simulink model "WiperSystem"  (R2023b)
settings: Solver=VariableStepAuto  StartTime=0.0  StopTime=20  RelTol=1e-3
libraries: simulink x6
settings Model: Creator=SEIF  LastModifiedBy=SEIF

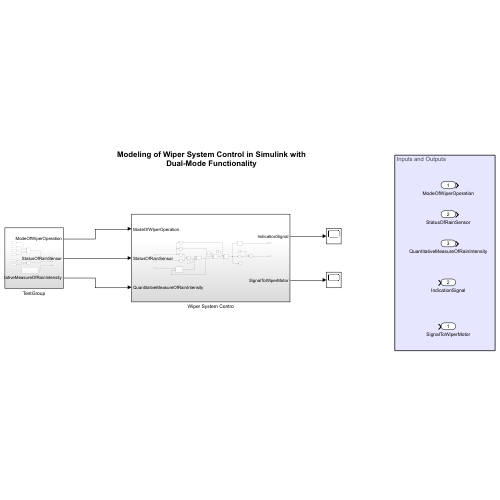
[thumbnail: Simulink's stored preview of the top-level diagram]
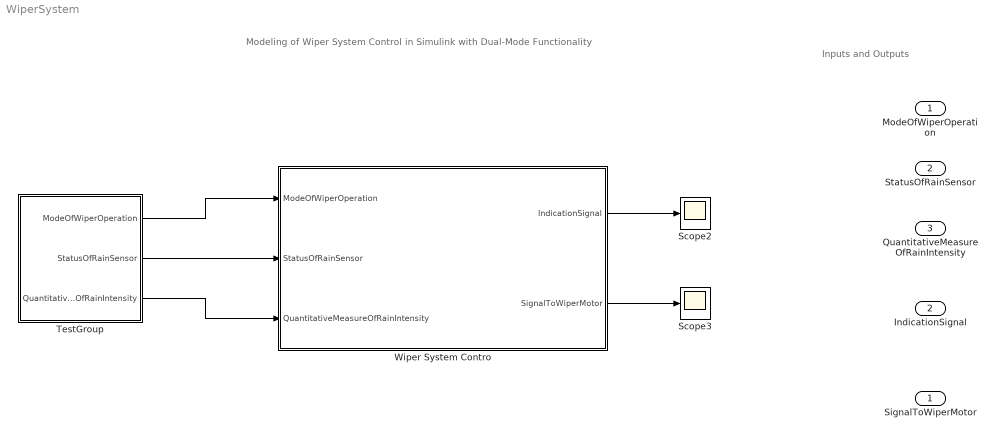
== system WiperSystem ==
  note: Inputs and Outputs
  note: Modeling of Wiper System Control in Simulink with Dual-Mode Functionality
  ModeOfWiperOperation : Inport
  StatusOfRainSensor : Inport  Port=2
  "QuantitativeMeasureOfRainIntensity " : Inport  Port=3
  Scope2 : Scope
  Scope3 : Scope
  TestGroup : Subsystem
  Wiper System Contro : Subsystem
  SignalToWiperMotor : Outport
  IndicationSignal : Outport  Port=2
  wires:
  TestGroup/3(QuantitativeMeasureOfRainIntensity) -> Wiper System Contro/3("QuantitativeMeasureOfRainIntensity ")
  TestGroup/2(StatusOfRainSensor) -> Wiper System Contro/2(StatusOfRainSensor)
  TestGroup/1(ModeOfWiperOperation) -> Wiper System Contro/1(ModeOfWiperOperation)
  Wiper System Contro/1(IndicationSignal) -> Scope2/1
  Wiper System Contro/2(SignalToWiperMotor) -> Scope3/1

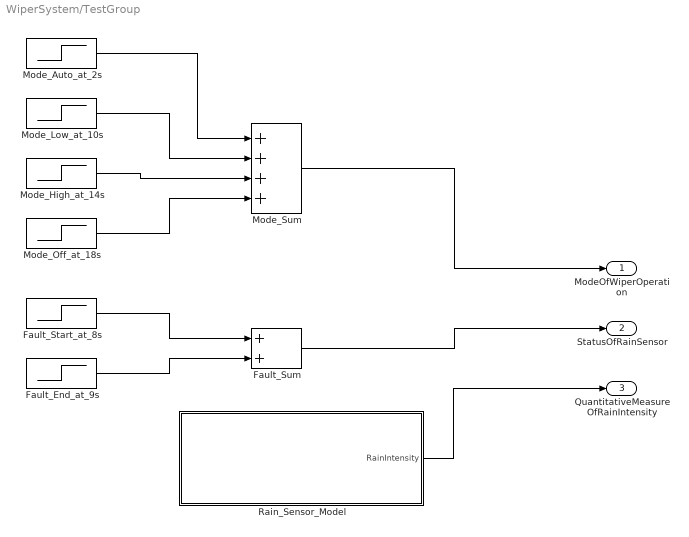
== system WiperSystem/TestGroup ==
  Fault_End_at_9s : Step  Time=9  After=-1  SampleTime=0.001
  Fault_Start_at_8s : Step  Time=8  SampleTime=0.001
  Fault_Sum : Sum
  Mode_Auto_at_2s : Step  Time=2  SampleTime=0.001
  Mode_High_at_14s : Step  Time=14  SampleTime=0.001
  Mode_Low_at_10s : Step  Time=10  SampleTime=0.001
  Mode_Off_at_18s : Step  Time=18  After=-3  SampleTime=0.001
  Mode_Sum : Sum  Inputs=++++
  Rain_Sensor_Model : Subsystem
  ModeOfWiperOperation : Outport
  StatusOfRainSensor : Outport  Port=2
  QuantitativeMeasureOfRainIntensity : Outport  Port=3
  wires:
  Mode_Auto_at_2s/1 -> Mode_Sum/1
  Mode_High_at_14s/1 -> Mode_Sum/3
  Fault_Sum/1 -> StatusOfRainSensor/1
  Mode_Off_at_18s/1 -> Mode_Sum/4
  Fault_Start_at_8s/1 -> Fault_Sum/1
  Mode_Sum/1 -> ModeOfWiperOperation/1
  Fault_End_at_9s/1 -> Fault_Sum/2
  Mode_Low_at_10s/1 -> Mode_Sum/2
  Rain_Sensor_Model/1(RainIntensity) -> QuantitativeMeasureOfRainIntensity/1

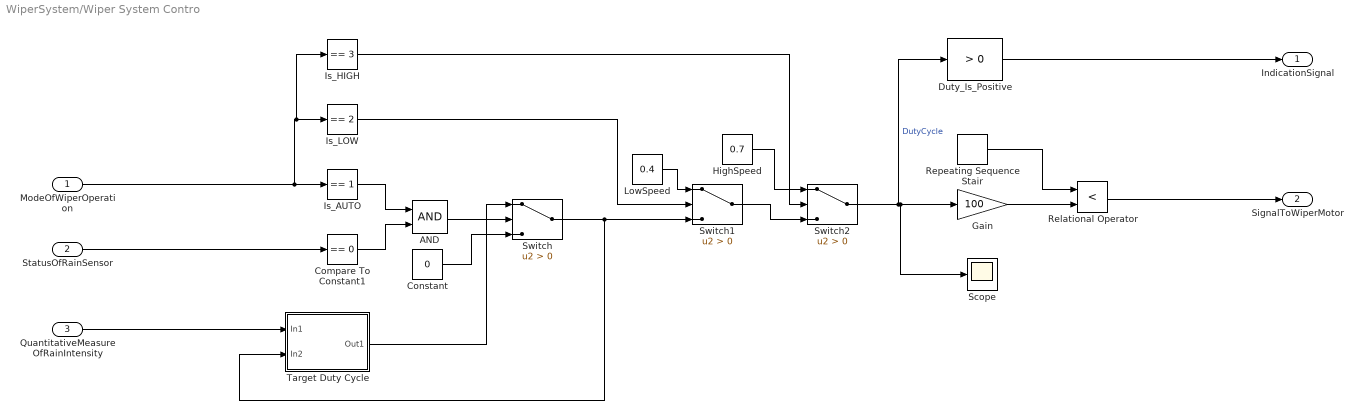
== system WiperSystem/Wiper System Contro ==
  ModeOfWiperOperation : Inport
  StatusOfRainSensor : Inport  Port=2
  "QuantitativeMeasureOfRainIntensity " : Inport  Port=3
  AND : Logic  AllPortsSameDT=off  OutDataTypeStr=boolean
  Compare To Constant1 : simulink/Logic and Bit Operations/Compare To Constant  relop===  const=0  OutDataTypeStr=boolean
  Constant : Constant  Value=0
  Duty_Is_Positive : simulink/Logic and Bit Operations/Compare To Constant  relop=>  const=0  OutDataTypeStr=boolean
  Gain : Gain  Gain=100
  HighSpeed : Constant  Value=0.7
  Is_AUTO : simulink/Logic and Bit Operations/Compare To Constant  relop===  const=1  OutDataTypeStr=boolean
  Is_HIGH : simulink/Logic and Bit Operations/Compare To Constant  relop===  const=3  OutDataTypeStr=boolean
  Is_LOW : simulink/Logic and Bit Operations/Compare To Constant  relop===  const=2  OutDataTypeStr=boolean
  LowSpeed : Constant  Value=0.4
  Relational Operator : RelationalOperator  Operator=<  OutDataTypeStr=boolean  RndMeth=Simplest  InputSameDT=off
  Repeating Sequence Stair : simulink/Sources/Repeating Sequence Stair  OutValues=0:99  tsamp=0.001  OutMin=[]  OutMax=[]  OutDataTypeStr=double  OutputDataTypeScalingMode=double  OutDataType=fixdt(0,8)  ConRadixGroup=Best Precision: Vector-wise  OutScaling=2^-12
  Scope : Scope
  Switch : Switch  Criteria=u2 > Threshold  SaturateOnIntegerOverflow=off  InputSameDT=off
  Switch1 : Switch  Criteria=u2 > Threshold  SaturateOnIntegerOverflow=off  InputSameDT=off
  Switch2 : Switch  Criteria=u2 > Threshold  SaturateOnIntegerOverflow=off  InputSameDT=off
  Target Duty Cycle : Subsystem
  IndicationSignal : Outport
  SignalToWiperMotor : Outport  Port=2
  wires:
  Repeating Sequence Stair/1 -> Relational Operator/1
  Switch2/1 -> Scope/1, Gain/1, Duty_Is_Positive/1  "DutyCycle"
  ModeOfWiperOperation/1 -> Is_HIGH/1, Is_LOW/1, Is_AUTO/1
  Is_AUTO/1 -> AND/1
  Switch1/1 -> Switch2/3
  Target Duty Cycle/1(Out1) -> Switch/1
  Constant/1 -> Switch/3
  Compare To Constant1/1 -> AND/2
  "QuantitativeMeasureOfRainIntensity "/1 -> Target Duty Cycle/1(In1)
  Gain/1 -> Relational Operator/2
  Switch/1 -> Target Duty Cycle/2(In2), Switch1/3
  AND/1 -> Switch/2
  LowSpeed/1 -> Switch1/1
  Is_LOW/1 -> Switch1/2
  HighSpeed/1 -> Switch2/1
  Is_HIGH/1 -> Switch2/2
  StatusOfRainSensor/1 -> Compare To Constant1/1
  Relational Operator/1 -> SignalToWiperMotor/1
  Duty_Is_Positive/1 -> IndicationSignal/1

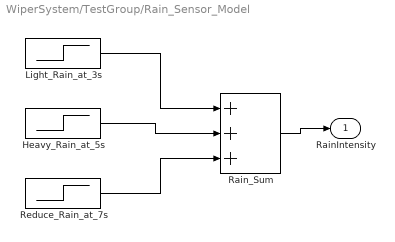
== system WiperSystem/TestGroup/Rain_Sensor_Model ==
  Heavy_Rain_at_5s : Step  Time=5  After=50  SampleTime=0.001
  Light_Rain_at_3s : Step  Time=3  After=20  SampleTime=0.001
  Rain_Sum : Sum  Inputs=+++
  Reduce_Rain_at_7s : Step  Time=7  After=-40  SampleTime=0.001
  RainIntensity : Outport
  wires:
  Light_Rain_at_3s/1 -> Rain_Sum/1
  Heavy_Rain_at_5s/1 -> Rain_Sum/2
  Reduce_Rain_at_7s/1 -> Rain_Sum/3
  Rain_Sum/1 -> RainIntensity/1

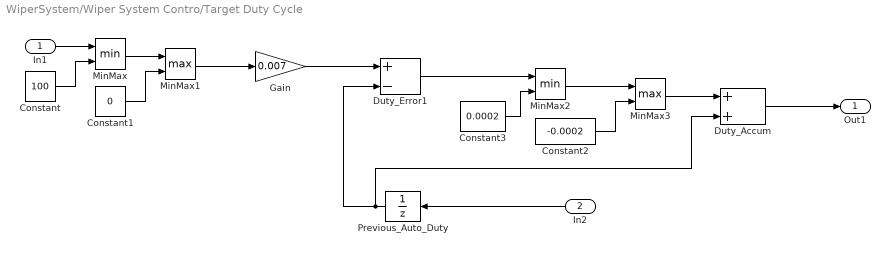
== system WiperSystem/Wiper System Contro/Target Duty Cycle ==
  In1 : Inport
  In2 : Inport  Port=2
  Constant : Constant  Value=100
  Constant1 : Constant  Value=0
  Constant2 : Constant  Value=-0.0002
  Constant3 : Constant  Value=0.0002
  Duty_Accum : Sum
  Duty_Error1 : Sum  Inputs=+-
  Gain : Gain  Gain=0.007
  MinMax : MinMax  Inputs=2
  MinMax1 : MinMax  Function=max  Inputs=2
  MinMax2 : MinMax  Inputs=2
  MinMax3 : MinMax  Function=max  Inputs=2
  Previous_Auto_Duty : UnitDelay  SampleTime=0.001  HasFrameUpgradeWarning=on
  Out1 : Outport
  wires:
  In1/1 -> MinMax/1
  Constant1/1 -> MinMax1/2
  Constant/1 -> MinMax/2
  MinMax/1 -> MinMax1/1
  MinMax1/1 -> Gain/1
  Gain/1 -> Duty_Error1/1
  Previous_Auto_Duty/1 -> Duty_Accum/2, Duty_Error1/2
  Duty_Error1/1 -> MinMax2/1
  Constant2/1 -> MinMax3/2
  Constant3/1 -> MinMax2/2
  MinMax2/1 -> MinMax3/1
  MinMax3/1 -> Duty_Accum/1
  Duty_Accum/1 -> Out1/1
  In2/1 -> Previous_Auto_Duty/1
